simulink model "untitled"  (R2024a)
settings: Solver=VariableStepAuto  StartTime=0.0  StopTime=10.0  RelTol=1e-3
undefined symbols (not defined in the file or in its folder): motor, motorDriver
settings Model: Creator=Marko  LastModifiedBy=Marko

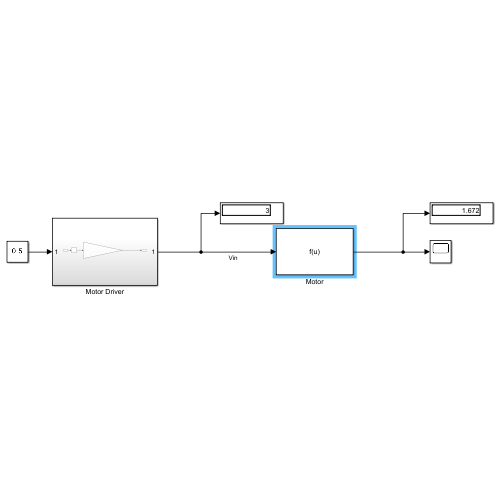
[thumbnail: Simulink's stored preview of the top-level diagram]
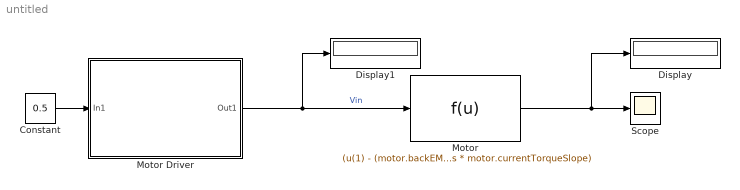
== system untitled ==
  Constant : Constant  Value=0.5
  Display : Display
  Display1 : Display
  Motor : Fcn  Expr=(u(1) - (motor.backEMFConstantVPerRad * (motor.noLoadSpeedRPM * 2 * pi / 60) + motor.noLoadCurrentA * motor.resistanceOhms)) / (-motor.backEMFConstantVPerRad * motor.speedTorqueSlope + motor.resistanceOhms * motor.currentTorqueSlope)
  Motor Driver : Subsystem
  Scope : Scope
  wires:
  Motor Driver/1(Out1) -> Display1/1, Motor/1  "Vin"
  Motor/1 -> Display/1, Scope/1
  Constant/1 -> Motor Driver/1(In1)

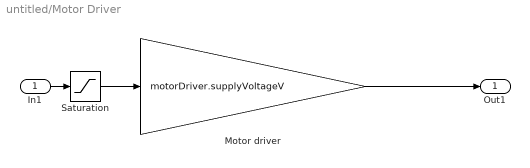
== system untitled/Motor Driver ==
  In1 : Inport
  Motor driver : Gain  Gain=motorDriver.supplyVoltageV
  Saturation : Saturate  UpperLimit=1  LowerLimit=0
  Out1 : Outport
  wires:
  Saturation/1 -> Motor driver/1
  In1/1 -> Saturation/1
  Motor driver/1 -> Out1/1
